simulink model "scheme_L2"  (R2026b)
settings: Solver=ode45  MaxStep=0.001  RelTol=1e-6  AbsTol=1e-8
settings Model: Creator=ALIENWARE  LastModifiedBy=Sofia
settings RTWCC: DLArmComputeVersion=19.05

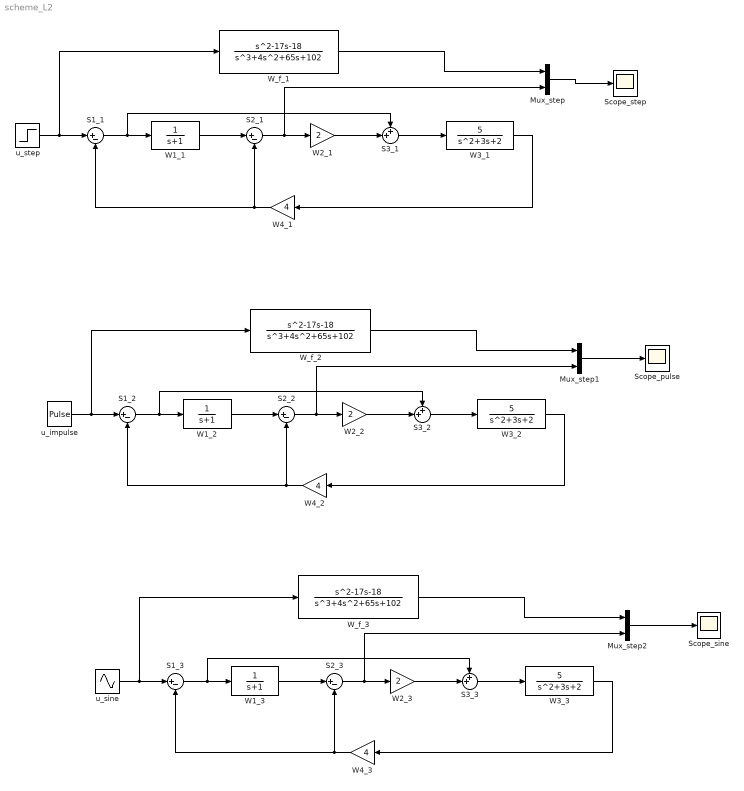
== system scheme_L2 ==
  Mux_step : Mux  Inputs=2
  Mux_step1 : Mux  Inputs=2
  Mux_step2 : Mux  Inputs=2
  S1_1 : Sum  Inputs=|+-
  S1_2 : Sum  Inputs=|+-
  S1_3 : Sum  Inputs=|+-
  S2_1 : Sum  Inputs=|+-
  S2_2 : Sum  Inputs=|+-
  S2_3 : Sum  Inputs=|+-
  S3_1 : Sum  Inputs=++|
  S3_2 : Sum  Inputs=++|
  S3_3 : Sum  Inputs=++|
  Scope_pulse : Scope
      settings: ActiveDisplayYMinimum=-2.28853905042628  ActiveDisplayYMaximum=1.7484332176566575  YLabel=y(t)
  Scope_sine : Scope
      settings: ActiveDisplayYMinimum=-0.27511635864621092  ActiveDisplayYMaximum=0.27260570502078935  YLabel=y(t)  DataLoggingVariableName=ScopeData2
  Scope_step : Scope
      settings: ActiveDisplayYMinimum=-0.49851531764738577  ActiveDisplayYMaximum=0.08217198651413303  YLabel=y(t)
  W1_1 : TransferFcn  Denominator=[1 1]
  W1_2 : TransferFcn  Denominator=[1 1]
  W1_3 : TransferFcn  Denominator=[1 1]
  W2_1 : Gain  Gain=2
  W2_2 : Gain  Gain=2
  W2_3 : Gain  Gain=2
  W3_1 : TransferFcn  Numerator=[5]  Denominator=[1 3 2]
  W3_2 : TransferFcn  Numerator=[5]  Denominator=[1 3 2]
  W3_3 : TransferFcn  Numerator=[5]  Denominator=[1 3 2]
  W4_1 : Gain  Gain=4
  W4_2 : Gain  Gain=4
  W4_3 : Gain  Gain=4
  W_f_1 : TransferFcn  Numerator=[1 -17 -18]  Denominator=[1 4 65 102]
  W_f_2 : TransferFcn  Numerator=[1 -17 -18]  Denominator=[1 4 65 102]
  W_f_3 : TransferFcn  Numerator=[1 -17 -18]  Denominator=[1 4 65 102]
  u_impulse : DiscretePulseGenerator  PulseType=Time based  Amplitude=100  Period=20  PulseWidth=0.05  PhaseDelay=1
  u_sine : Sin  SampleTime=0
  u_step : Step  SampleTime=0
  wires:
  u_step/1 -> W_f_1/1, S1_1/1
  S1_1/1 -> S3_1/1, W1_1/1
  W1_1/1 -> S2_1/1
  S2_1/1 -> W2_1/1, Mux_step/2
  W2_1/1 -> S3_1/2
  S3_1/1 -> W3_1/1
  W3_1/1 -> W4_1/1
  W4_1/1 -> S2_1/2, S1_1/2
  Mux_step/1 -> Scope_step/1
  W_f_1/1 -> Mux_step/1
  S1_2/1 -> S3_2/1, W1_2/1
  W4_2/1 -> S2_2/2, S1_2/2
  W_f_2/1 -> Mux_step1/1
  W2_2/1 -> S3_2/2
  S2_2/1 -> W2_2/1, Mux_step1/2
  W1_2/1 -> S2_2/1
  Mux_step1/1 -> Scope_pulse/1
  u_impulse/1 -> W_f_2/1, S1_2/1
  S3_2/1 -> W3_2/1
  W3_2/1 -> W4_2/1
  S1_3/1 -> S3_3/1, W1_3/1
  W4_3/1 -> S2_3/2, S1_3/2
  W_f_3/1 -> Mux_step2/1
  W2_3/1 -> S3_3/2
  S2_3/1 -> W2_3/1, Mux_step2/2
  W1_3/1 -> S2_3/1
  u_sine/1 -> W_f_3/1, S1_3/1
  S3_3/1 -> W3_3/1
  W3_3/1 -> W4_3/1
  Mux_step2/1 -> Scope_sine/1
